simulink model "Robot_model_Turnrate_Control_ZOH_2025b"  (R2026a)
settings: Solver=VariableStepAuto  StopTime=10
values from neighbouring files (symbols this model uses):
  B = D * L    (= 9.682e-08)    [measurements.m]    (also in run_simulink.m = 0.15; run_simulink_PI_Controller.m = 0.15; run_simulink_turnrate_Controller.m = 0.15; run_simulink_turnrate_Controller_Heading.m = 0.15)
  D = 0.0000188    (= 1.88e-05)    [measurements.m]    (also in motor_model_m.m = 5e-05; run_simulink.m = 5e-05; run_simulink_PI_Controller.m = 5e-05; run_simulink_turnrate_Controller.m = 5e-05)
  J = -b / a    (= 2.25042607204e-06)    [measurements.m]    (also in motor_model_m.m = 5.56231644013e-06; run_simulink.m = 5.56231644013e-06; run_simulink_PI_Controller.m = 5.56231644013e-06; run_simulink_turnrate_Controller.m = 5.56231644013e-06)
  Kb = Kt    (= 0.009)    [motor_model_m.m]    (also in run_simulink.m; run_simulink_PI_Controller.m; run_simulink_turnrate_Controller.m; run_simulink_turnrate_Controller_Heading.m)
  Kp = 0.1202    [motor_model_m.m]    (also in run_simulink.m; run_simulink_PI_Controller.m; run_simulink_turnrate_Controller.m; run_simulink_turnrate_Controller_Heading.m)
  Kpt = 3    [run_simulink_turnrate_Controller.m]    (also in run_simulink_turnrate_Controller_Heading.m)
  Kt = 0.009    [motor_model_m.m]    (also in run_simulink.m; run_simulink_PI_Controller.m; run_simulink_turnrate_Controller.m; run_simulink_turnrate_Controller_Heading.m)
  L = 5.15e-3    (= 0.00515)    [measurements.m]    (also in motor_model_m.m = 0.0045; run_simulink.m = 0.0045; run_simulink_PI_Controller.m = 0.0045; run_simulink_turnrate_Controller.m = 0.0045)
  mesDelay = 10*1e-3    (= 0.01)    [run_simulink.m]    (also in run_simulink_PI_Controller.m; run_simulink_turnrate_Controller.m; run_simulink_turnrate_Controller_Heading.m)
  R = 4.29    [measurements.m]    (also in motor_model_m.m; run_simulink.m; run_simulink_PI_Controller.m; run_simulink_turnrate_Controller.m)
  r2m = wheelRadius/gear    (= 0.00309917355372)    [motor_model_m.m]    (also in run_simulink.m; run_simulink_PI_Controller.m; run_simulink_turnrate_Controller.m; run_simulink_turnrate_Controller_Heading.m)
  taui_t = 0.4    [run_simulink_turnrate_Controller.m]    (also in run_simulink_turnrate_Controller_Heading.m)
  Ti = 0.0685    [motor_model_m.m]    (also in run_simulink_PI_Controller.m; run_simulink_turnrate_Controller.m; run_simulink_turnrate_Controller_Heading.m)
  Ts = 0.01    [run_simulink.m]    (also in run_simulink_PI_Controller.m; run_simulink_turnrate_Controller.m; run_simulink_turnrate_Controller_Heading.m)
settings Model: Creator=chr  LastModifiedBy=mirmu

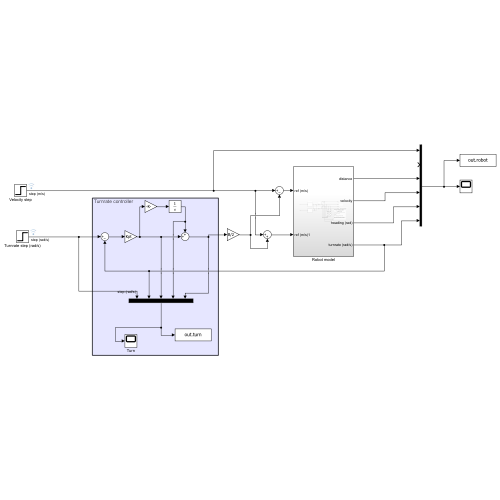
[thumbnail: Simulink's stored preview of the top-level diagram]
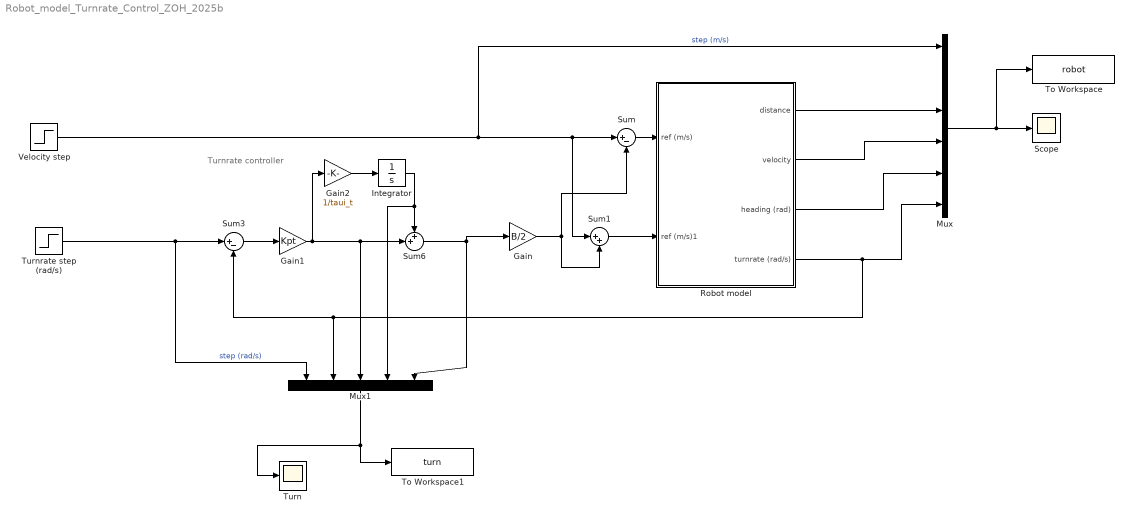
== system Robot_model_Turnrate_Control_ZOH_2025b ==
  note: Turnrate controller
  Gain : Gain  Gain=B/2
  Gain1 : Gain  Gain=Kpt
  Gain2 : Gain  Gain=1/taui_t
  Integrator : Integrator
  Mux : Mux  Inputs=6
  Mux1 : Mux  Inputs=5
  Robot model : Subsystem
  Scope : Scope
      settings: ActiveDisplayYMinimum=0.046275084880073314  ActiveDisplayYMaximum=0.2985926907550987  DataLoggingVariableName=ScopeData2
  Sum : Sum  Inputs=|+-
  Sum1 : Sum  Inputs=|++
  Sum3 : Sum  Inputs=|+-
  Sum6 : Sum  Inputs=++|
  To Workspace : ToWorkspace  VariableName=robot  SampleTime=-1
  To Workspace1 : ToWorkspace  VariableName=turn  SampleTime=-1
  Turn : Scope
      settings: ActiveDisplayYMinimum=-1.25330333501178  ActiveDisplayYMaximum=3.2010990636697292  DataLoggingVariableName=ScopeData3
  Turnrate step (rad/s) : Step  Time=0.5  SampleTime=0
  Velocity step : Step  Time=0.3  FinalValue=0.2  SampleTime=0
  wires:
  Gain/1 -> Sum/2, Sum1/2
  Velocity step/1 -> Mux/1, Sum1/1, Sum/1  "step (m/s)"
  Sum/1 -> Robot model/1(ref (m/s))
  Sum1/1 -> Robot model/2(ref (m/s)1)
  Robot model/1(distance) -> Mux/3
  Robot model/2(velocity) -> Mux/4
  Robot model/3(heading (rad)) -> Mux/5
  Robot model/4(turnrate (rad/s)) -> Mux1/2, Sum3/2, Mux/6
  Mux/1 -> To Workspace/1, Scope/1
  Turnrate step (rad/s)/1 -> Mux1/1, Sum3/1  "step (rad/s)"
  Sum3/1 -> Gain1/1
  Gain1/1 -> Gain2/1, Mux1/3, Sum6/2
  Gain2/1 -> Integrator/1
  Integrator/1 -> Mux1/4, Sum6/1
  Sum6/1 -> Gain/1, Mux1/5
  Mux1/1 -> To Workspace1/1, Turn/1

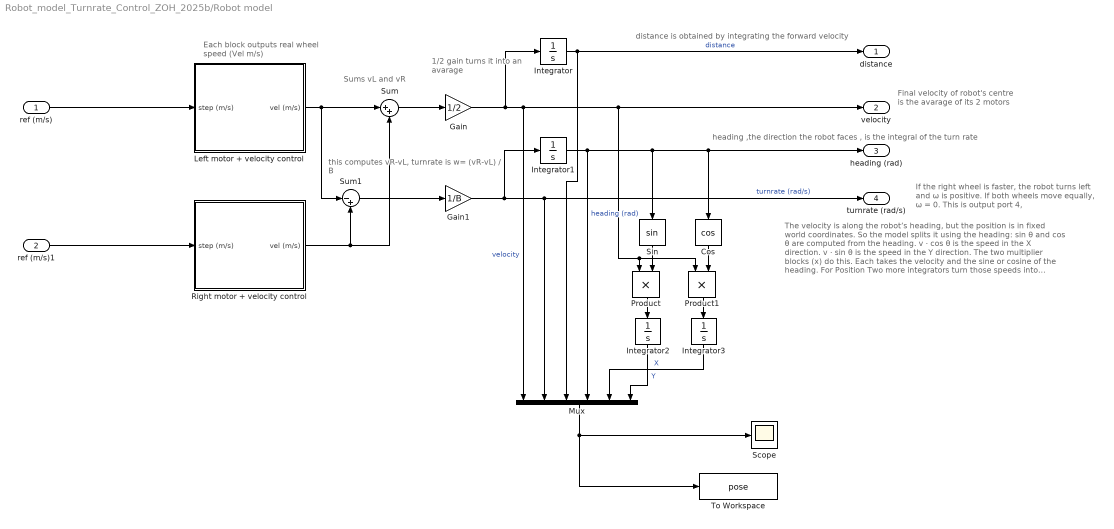
== system Robot_model_Turnrate_Control_ZOH_2025b/Robot model ==
  note: The velocity is along the robot’s heading, but the position is in fixed world coordinates. So the model splits it using the heading:
      | sin θ and cos θ are computed from the heading.
      | v · cos θ is the speed in the X direction.
      | v · sin θ is the speed in the Y direction.
      | The two multiplier blocks (x) do this. Each takes the velocity and the sine or cosine of the heading.
      | For Position
      | Two more integrators turn those speeds into position:
      | X = ∫ v·cos θ dt and Y = ∫ v·sin θ dt
      | In the diagram, the sin path ends at the integrator labelled Y, and the cos path at the one labelled X. With θ = 0 the robot moves along +X, and a positive turn rate rotates it counter-clockwise.
  note: heading ,the direction the robot faces , is the integral of the turn rate
  note: distance is obtained by integrating the forward velocity
  note: If the right wheel is faster, the robot turns left and ω is positive. If both wheels move equally, ω = 0. This is output port 4,
  note: this computes vR-vL, turnrate is w= (vR-vL) / B
  note: Final velocity of robot's centre is the avarage of its 2 motors
  note: 1/2 gain turns it into an avarage
  note: Sums vL and vR
  note: Each block outputs real wheel speed (Vel m/s)
  ref (m/s) : Inport
  ref (m/s)1 : Inport  Port=2
  Cos : Trigonometry  Operator=cos
  Gain : Gain  Gain=1/2
  Gain1 : Gain  Gain=1/B
  Integrator{,1..3} (4 alike) : Integrator
  "Left motor + velocity control " : Subsystem
  Mux : Mux  Inputs=6
  Product : Product
  Product1 : Product
  "Right motor + velocity control " : Subsystem
  Scope : Scope
      settings: ActiveDisplayYMinimum=-0.16521318377244509  ActiveDisplayYMaximum=1.5090083830749093
  Sin : Trigonometry
  Sum : Sum  Inputs=|++
  Sum1 : Sum  Inputs=|-+
  To Workspace : ToWorkspace  VariableName=pose  SaveFormat=Timeseries  SampleTime=-1
  distance : Outport
  velocity : Outport  Port=2
  heading (rad) : Outport  Port=3
  turnrate (rad/s) : Outport  Port=4
  wires:
  Gain/1 -> Integrator/1, Mux/1, velocity/1, Product1/1, Product/1  "velocity"
  "Right motor + velocity control "/1(vel (m/s)) -> Sum/2, Sum1/2
  Mux/1 -> To Workspace/1, Scope/1
  Gain1/1 -> Integrator1/1, turnrate (rad/s)/1, Mux/2  "turnrate (rad/s)"
  Integrator3/1 -> Mux/5  "X"
  ref (m/s)1/1 -> "Right motor + velocity control "/1(step (m/s))
  Integrator/1 -> distance/1, Mux/3  "distance"
  "Left motor + velocity control "/1(vel (m/s)) -> Sum/1, Sum1/1
  ref (m/s)/1 -> "Left motor + velocity control "/1(step (m/s))
  Integrator1/1 -> Sin/1, heading (rad)/1, Cos/1, Mux/4  "heading (rad)"
  Sum1/1 -> Gain1/1
  Sum/1 -> Gain/1
  Product/1 -> Integrator2/1
  Cos/1 -> Product1/2
  Integrator2/1 -> Mux/6  "Y"
  Sin/1 -> Product/2
  Product1/1 -> Integrator3/1

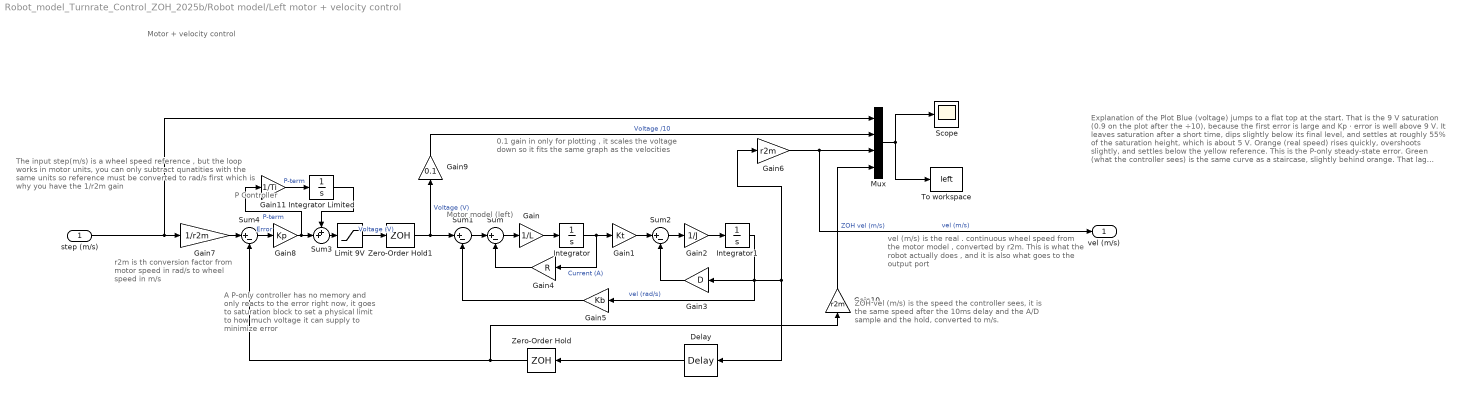
== system Robot_model_Turnrate_Control_ZOH_2025b/Robot model/Left motor + velocity control  ==
  note: Explanation of the Plot
      |
      | Blue (voltage) jumps to a flat top at the start. That is the 9 V saturation (0.9 on the plot after the ÷10), because the first error is large and Kp · error is well above 9 V. It leaves saturation after a short time, dips slightly below its final level, and settles at roughly 55% of the saturation height, which is about 5 V.
      |
      | Orange (real speed) rises quickly, overshoots slightly, and settles below the yellow reference. This is the P-only steady-state error.
      |
      | Green (what the controller sees) is the same curve as a staircase, slightly behind orange. That lag comes from the 10 ms delay plus the sample and hold.
  note: ZOH vel (m/s) is the speed the controller sees, it is the same speed after the 10ms delay and the A/D sample and the hold, converted to m/s.
  note: vel (m/s) is the real . continuous wheel speed from the motor model , converted by r2m. This is what the robot actually does , and it is also what goes to the output port
  note: 0.1 gain in only for plotting , it scales the voltage down so it fits the same graph as the velocities
  note: A P-only controller has no memory and only reacts to the error right now, it goes to saturation block to set a physical limit to how much voltage it can supply to minimize error
  note: The input step(m/s) is a wheel speed reference , but the loop works in motor units, you can only subtract qunatities with the same units so reference must be converted to rad/s first which is why you have the 1/r2m gain
  note: r2m is th conversion factor from motor speed in rad/s to wheel speed in m/s
  note: Motor + velocity control
  note: P Controller
  note: Motor model (left)
  step (m/s) : Inport
  Delay : TransportDelay  DelayTime=mesDelay
  Gain : Gain  Gain=1/L
  Gain1 : Gain  Gain=Kt
  Gain10 : Gain  Gain=r2m
  Gain11 : Gain  Gain=1/Ti
  Gain2 : Gain  Gain=1/J
  Gain3 : Gain  Gain=D
  Gain4 : Gain  Gain=R
  Gain5 : Gain  Gain=Kb
  Gain6 : Gain  Gain=r2m
  Gain7 : Gain  Gain=1/r2m
  Gain8 : Gain  Gain=Kp
  Gain9 : Gain  Gain=0.1
  Integrator : Integrator
  Integrator Limited : Integrator  LimitOutput=on  UpperSaturationLimit=8  LowerSaturationLimit=-8
  Integrator1 : Integrator
  Limit 9V : Saturate  UpperLimit=9  LowerLimit=-9
  Mux : Mux
  Scope : Scope
      settings: ActiveDisplayYMinimum=-0.17273093002303094  ActiveDisplayYMaximum=0.33208426078463232
  Sum{,1..2,4} (4 alike) : Sum  Inputs=|+-
  Sum3 : Sum  Inputs=++|
  To workspace : ToWorkspace  VariableName=left  SaveFormat=Timeseries  SampleTime=-1
  Zero-Order Hold : ZeroOrderHold  SampleTime=Ts
  Zero-Order Hold1 : ZeroOrderHold  SampleTime=Ts
  vel (m/s) : Outport
  wires:
  Gain10/1 -> Mux/4  "ZOH vel (m/s)"
  Gain/1 -> Integrator/1
  Integrator1/1 -> Gain3/1, Gain5/1, Gain6/1, Delay/1  "vel (rad/s)"
  Gain7/1 -> Sum4/1
  Integrator/1 -> Gain4/1, Gain1/1  "Current (A)"
  step (m/s)/1 -> Mux/1, Gain7/1
  Gain5/1 -> Sum1/2
  Sum4/1 -> Gain8/1  "Error"
  Sum/1 -> Gain/1
  Gain2/1 -> Integrator1/1
  Sum1/1 -> Sum/1
  Mux/1 -> Scope/1, To workspace/1
  Sum2/1 -> Gain2/1
  Gain3/1 -> Sum2/2
  Gain1/1 -> Sum2/1
  Gain6/1 -> vel (m/s)/1, Mux/3  "vel (m/s)"
  Zero-Order Hold/1 -> Gain10/1, Sum4/2
  Limit 9V/1 -> Zero-Order Hold1/1  "Voltage (V)"
  Zero-Order Hold1/1 -> Sum1/1, Gain9/1  "Voltage (V)"
  Delay/1 -> Zero-Order Hold/1
  Gain4/1 -> Sum/2
  Gain9/1 -> Mux/2  "Voltage /10"
  Gain8/1 -> Gain11/1, Sum3/2  "P-term"
  Sum3/1 -> Limit 9V/1
  Gain11/1 -> Integrator Limited/1  "P-term"
  Integrator Limited/1 -> Sum3/1

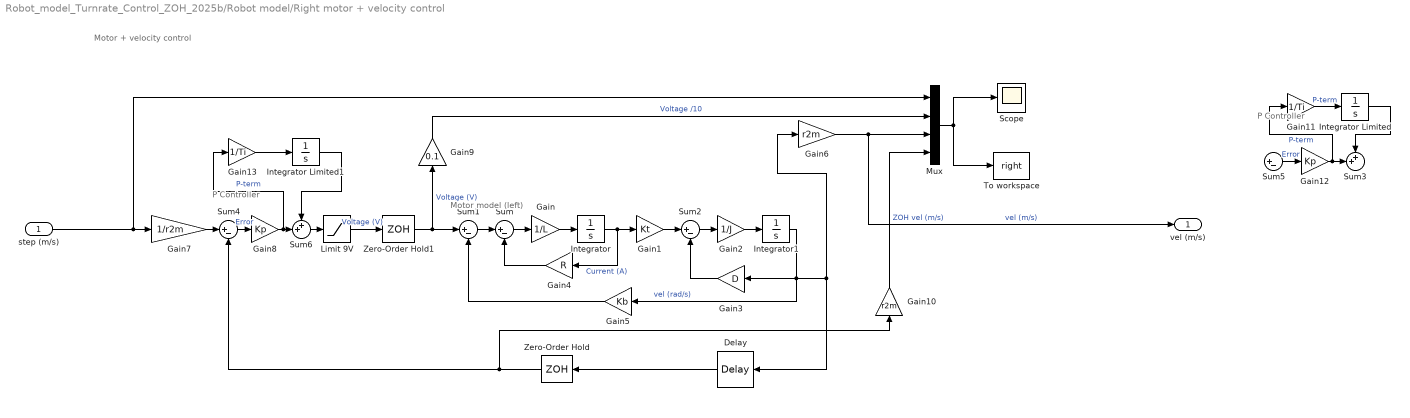
== system Robot_model_Turnrate_Control_ZOH_2025b/Robot model/Right motor + velocity control  ==
  note: Motor + velocity control
  note: Motor model (left)
  note: P Controller
  note: P Controller
  step (m/s) : Inport
  Delay : TransportDelay  DelayTime=mesDelay
  Gain : Gain  Gain=1/L
  Gain1 : Gain  Gain=Kt
  Gain10 : Gain  Gain=r2m
  Gain11 : Gain  Gain=1/Ti
  Gain12 : Gain  Gain=Kp
  Gain13 : Gain  Gain=1/Ti
  Gain2 : Gain  Gain=1/J
  Gain3 : Gain  Gain=D
  Gain4 : Gain  Gain=R
  Gain5 : Gain  Gain=Kb
  Gain6 : Gain  Gain=r2m
  Gain7 : Gain  Gain=1/r2m
  Gain8 : Gain  Gain=Kp
  Gain9 : Gain  Gain=0.1
  Integrator : Integrator
  Integrator Limited : Integrator  LimitOutput=on  UpperSaturationLimit=8  LowerSaturationLimit=-8
  Integrator Limited1 : Integrator  LimitOutput=on  UpperSaturationLimit=8  LowerSaturationLimit=-8
  Integrator1 : Integrator
  Limit 9V : Saturate  UpperLimit=9  LowerLimit=-9
  Mux : Mux
  Scope : Scope
      settings: ActiveDisplayYMinimum=0.0023805362037857547  ActiveDisplayYMaximum=0.64443672037004684
  Sum{,1..2,4..5} (5 alike) : Sum  Inputs=|+-
  Sum3 : Sum  Inputs=++|
  Sum6 : Sum  Inputs=++|
  To workspace : ToWorkspace  VariableName=right  SaveFormat=Timeseries  SampleTime=-1
  Zero-Order Hold : ZeroOrderHold  SampleTime=Ts
  Zero-Order Hold1 : ZeroOrderHold  SampleTime=Ts
  vel (m/s) : Outport
  wires:
  Gain9/1 -> Mux/2  "Voltage /10"
  Gain4/1 -> Sum/2
  Delay/1 -> Zero-Order Hold/1
  Zero-Order Hold1/1 -> Gain9/1, Sum1/1  "Voltage (V)"
  Limit 9V/1 -> Zero-Order Hold1/1  "Voltage (V)"
  Zero-Order Hold/1 -> Sum4/2, Gain10/1
  Gain6/1 -> Mux/3, vel (m/s)/1  "vel (m/s)"
  Gain1/1 -> Sum2/1
  Gain3/1 -> Sum2/2
  Sum2/1 -> Gain2/1
  Mux/1 -> To workspace/1, Scope/1
  Sum1/1 -> Sum/1
  Gain8/1 -> Sum6/2, Gain13/1  "P-term"
  Gain2/1 -> Integrator1/1
  Sum/1 -> Gain/1
  Sum4/1 -> Gain8/1  "Error"
  Gain5/1 -> Sum1/2
  step (m/s)/1 -> Gain7/1, Mux/1
  Integrator/1 -> Gain1/1, Gain4/1  "Current (A)"
  Gain7/1 -> Sum4/1
  Integrator1/1 -> Delay/1, Gain6/1, Gain5/1, Gain3/1  "vel (rad/s)"
  Gain/1 -> Integrator/1
  Gain10/1 -> Mux/4  "ZOH vel (m/s)"
  Gain11/1 -> Integrator Limited/1  "P-term"
  Gain12/1 -> Gain11/1, Sum3/2  "P-term"
  Sum5/1 -> Gain12/1  "Error"
  Integrator Limited/1 -> Sum3/1
  Gain13/1 -> Integrator Limited1/1
  Integrator Limited1/1 -> Sum6/1
  Sum6/1 -> Limit 9V/1
